simulink library "ConverterLibrary"  (R2026a)
settings: Solver=VariableStepAuto
undefined symbols (not defined in the file or in its folder): DiscIntNeverNeededParam, dspblkCoreblockFVToolHelper, gcbh, gridInverter
libraries: fl_lib x240, nesl_utility x221, ee_lib x208, slpidlib x28, eeGeneralControl x12, simulink x9, eeTransforms x4, simulink_extras x1, eePowerMeasurement x1
(part 15 of 30)

== system ConverterLibrary/Controller/Inverter-Based Resources/Grid-Forming Converter Controller/Grid Voltage Reactive Power Support/Modifying Reactive Power Reference/Changing the Power Reference/ActivePowerReference ==
  note: Ensure Pref sign is maintained
  Id : Inport
  Vd : Inport  Port=2
  Pref : Inport  Port=3
  Abs1 : Abs  SaturateOnIntegerOverflow=off
  Abs2 : Abs  SaturateOnIntegerOverflow=off
  Min : MinMax  Inputs=2
  Product : Product
  Product2 : Product
  Saturation : Saturate  UpperLimit=1  LowerLimit=-1
  Sign : Signum
  PrefNew : Outport
  wires:
  Saturation/1 -> PrefNew/1
  Vd/1 -> Product/2
  Abs2/1 -> Min/1
  Product2/1 -> Saturation/1
  Min/1 -> Product2/1
  Product/1 -> Abs2/1
  Abs1/1 -> Min/2
  Sign/1 -> Product2/2
  Id/1 -> Product/1
  Pref/1 -> Sign/1, Abs1/1

== system ConverterLibrary/Controller/Inverter-Based Resources/Grid-Forming Converter Controller/Grid Voltage Reactive Power Support/Modifying Reactive Power Reference/Changing the Power Reference/Estimate Id for Given Iq ==
  Iq : Inport
  Add Constant1 : Bias  Bias=1  SaturateOnIntegerOverflow=off
  Gain : Gain  Gain=-1
  Gain3 : Gain  Gain=0.9
  Sqrt : Sqrt
  Square : Math  Operator=square
  Id : Outport
  wires:
  Iq/1 -> Square/1
  Add Constant1/1 -> Sqrt/1
  Sqrt/1 -> Gain3/1
  Gain/1 -> Add Constant1/1
  Gain3/1 -> Id/1
  Square/1 -> Gain/1

== system ConverterLibrary/Controller/Inverter-Based Resources/Grid-Forming Converter Controller/Grid Voltage Reactive Power Support/Modifying Reactive Power Reference/Changing the Power Reference/EstimateIqForReactivePower ==
  note: Computing minimum reactive current as per GC0137
  Vmin : Inport
  Vd : Inport  Port=2
  Vs : Inport  Port=3
  Abs : Abs  SaturateOnIntegerOverflow=off
  Add : Sum
  Add Constant : Bias  Bias=1  SaturateOnIntegerOverflow=off
  GC0137 line slope : Gain  Gain=-1.4578
  Low Voltage Support : Subsystem
  Saturation : Saturate  UpperLimit=1  LowerLimit=0
  Iq : Outport
  wires:
  Low Voltage Support/1(Iqsupport) -> Add/1
  Vd/1 -> Low Voltage Support/2(Vd)
  Vmin/1 -> Low Voltage Support/1(Vin)
  Add Constant/1 -> Add/2
  Saturation/1 -> Iq/1
  Add/1 -> Saturation/1
  Vs/1 -> Abs/1
  GC0137 line slope/1 -> Add Constant/1
  Abs/1 -> GC0137 line slope/1

== system ConverterLibrary/Controller/Inverter-Based Resources/Grid-Forming Converter Controller/Grid Voltage Reactive Power Support/Modifying Reactive Power Reference/Changing the Power Reference/ReactivePowerReference ==
  Vd : Inport
  Iq : Inport  Port=2
  Compute Power : Product
  Constant : Constant  Value=0.3
  Gain2 : Gain  Gain=1.05
  Switch : Switch  Criteria=u2 > Threshold  Threshold=0.3  SaturateOnIntegerOverflow=off  InputSameDT=off
  QrefNew : Outport
  wires:
  Switch/1 -> Compute Power/1
  Vd/1 -> Switch/1, Switch/2
  Iq/1 -> Gain2/1
  Constant/1 -> Switch/3
  Gain2/1 -> Compute Power/2
  Compute Power/1 -> QrefNew/1

== system ConverterLibrary/Controller/Inverter-Based Resources/Grid-Forming Converter Controller/Measurement/Frequency Measurement/Frequency Measurement/If Action Subsystem ==
  V : Inport
  Time : Inport  Port=2
  Action Port : ActionPort
  Constant1 : Constant  Value=initialFrequency
  Delay : Delay  DelayLength=1
  Delay1 : Delay  DelayLength=1
  Frequency estimation : Subsystem  TreatAsAtomicUnit=on
  Hit Crossing : HitCross
  Switch : Switch  Criteria=u2 > Threshold  Threshold=1  SaturateOnIntegerOverflow=off  InputSameDT=off
  Freq : Outport
  wires:
  Switch/1 -> Freq/1
  Constant1/1 -> Switch/3
  Frequency estimation/1(f) -> Switch/1
  Time/1 -> Frequency estimation/3(k), Delay1/1, Switch/2
  Delay/1 -> Frequency estimation/2(sk-1)
  Hit Crossing/1 -> Frequency estimation/Trigger
  Delay1/1 -> Frequency estimation/4(k-1)
  V/1 -> Hit Crossing/1, Frequency estimation/1(sk), Delay/1

== system ConverterLibrary/Controller/Inverter-Based Resources/Grid-Forming Converter Controller/Measurement/Frequency Measurement/Frequency Measurement/If Action Subsystem1 ==
  Action Port : ActionPort
  Constant1 : Constant  Value=initialFrequency
  Out1 : Outport
  wires:
  Constant1/1 -> Out1/1

== system ConverterLibrary/Controller/Inverter-Based Resources/Grid-Forming Converter Controller/Measurement/Frequency Measurement/Frequency Measurement/Postive Sequence ==
  abc : Inport
  Complex to Real-Imag : ComplexToRealImag
  Demux : Demux  Outputs=3
  Symmetrical-Components Transform : eeTransforms/Symmetrical-Components Transform  PowerInvariant=off
      settings: LibrarySourceBlock=|
      | ee_sl_lib/Mathematical
      | Transforms/Symmetrical-Components
      | Transform
  Terminator : Terminator
  Terminator1 : Terminator
  Terminator2 : Terminator
  Transpose : Math  Operator=transpose
  posSeq : Outport
  wires:
  Demux/3 -> Terminator2/1
  Demux/2 -> Terminator1/1
  Complex to Real-Imag/2 -> Terminator/1
  abc/1 -> Transpose/1
  Demux/1 -> Complex to Real-Imag/1
  Complex to Real-Imag/1 -> posSeq/1
  Symmetrical-Components Transform/1 -> Demux/1
  Transpose/1 -> Symmetrical-Components Transform/1

== system ConverterLibrary/Controller/Inverter-Based Resources/Grid-Forming Converter Controller/Power Control/ActivePowerControl/vsmControl/Damping Frequency ==
  fref : Inport
  ConstantFreqReference : Subsystem  VariantControl=constFreq
  WithFrequencyMeasurement : Subsystem  VariantControl=freqMeas
  fmeas : Outport

== system ConverterLibrary/Controller/Non-Isolated DC-DC Converters/Non-Isolated DC-DC Controller/Loop Structure/DoubleLoop/Current Controller/PIContinuous ==
  error : Inport
  up : Inport  Port=2
  lo : Inport  Port=3
  PI Controller : slpidlib/PID Controller  Controller=PI  Form=Parallel  TimeDomain=Continuous-time  UseExternalTs=off  SampleTime=-1  IntegratorMethod=Forward Euler  FilterMethod=Forward Euler  ControllerParametersSource=internal  P=KpCurrent  I=KiCurrent  UseKiTs=off  D=0  UseExternalDerivativeSource=off  N=100  UseFilter=on  TunerSelectOption=Transfer Function Based (PID Tuner App)  InitialConditionSource=internal  InitialConditionForIntegrator=0  InitialConditionForFilter=0  DifferentiatorICPrevScaledInput=0  ExternalReset=none  TrackingMode=off  Kt=1  LimitOutput=on  SatLimitsSource=external  UpperSaturationLimit=1  LowerSaturationLimit=-1  LinearizeAsGain=on  AntiWindupMode=clamping  Kb=1  LimitIntegrator=on  UpperIntegratorSaturationLimit=dutyTrimSpan  LowerIntegratorSaturationLimit=-dutyTrimSpan  POutMin=[]  POutMax=[]  IOutMin=[]  IOutMax=[]  DOutMin=[]  DOutMax=[]  NOutMin=[]  NOutMax=[]  SumOutMin=[]  SumOutMax=[]  SaturationOutMin=[]  SaturationOutMax=[]  PParamMin=[]  PParamMax=[]  IParamMin=[]  IParamMax=[]  DParamMin=[]  DParamMax=[]  NParamMin=[]  NParamMax=[]  KbParamMin=[]  KbParamMax=[]  KtParamMin=[]  KtParamMax=[]  KbOutMin=[]  KbOutMax=[]  KtOutMin=[]  KtOutMax=[]  IntegratorOutMin=[]  IntegratorOutMax=[]  FilterOutMin=[]  FilterOutMax=[]  SumI1OutMin=[]  SumI1OutMax=[]  SumI2OutMin=[]  SumI2OutMax=[]  SumI3OutMin=[]  SumI3OutMax=[]  SumI4OutMin=[]  SumI4OutMax=[]  SumDOutMin=[]  SumDOutMax=[]  DifferentiatorOutMin=[]  DifferentiatorOutMax=[]  FilterDiffOutCoefMin=[]  FilterDiffOutCoefMax=[]  ReciprocalOutMin=[]  ReciprocalOutMax=[]  SumDenOutMin=[]  SumDenOutMax=[]  SumNumOutMin=[]  SumNumOutMax=[]  DivideOutMin=[]  DivideOutMax=[]  UdiffTsProdOutMin=[]  UdiffTsProdOutMax=[]  NTsProdOutMin=[]  NTsProdOutMax=[]  UintegralTsProdOutMin=[]  UintegralTsProdOutMax=[]  UngainTsProdOutMin=[]  UngainTsProdOutMax=[]  ClampingZeroOutDataTypeStr=Inherit: Inherit via back propagation  ClampingZeroOutMin=[]  ClampingZeroOutMax=[]  FilterDenConstantOutDataTypeStr=Inherit: Inherit via back propagation  FilterDenConstantOutMin=[]  FilterDenConstantOutMax=[]  PCopyOutDataTypeStr=Inherit: Inherit via back propagation  PCopyOutMin=[]  PCopyOutMax=[]  NCopyOutDataTypeStr=Inherit: Inherit via back propagation  NCopyOutMin=[]  NCopyOutMax=[]  IntegratorContinuousStateAttributes=''  IntegratorStateMustResolveToSignalObject=off  IntegratorRTWStateStorageClass=Auto  FilterContinuousStateAttributes=''  FilterStateMustResolveToSignalObject=off  FilterRTWStateStorageClass=Auto  ParallelPVariant=InternalParameters  IdealPVariant=Disabled  IVariant=InternalParameters  DVariant=Disabled  IntegratorVariant=Continuous  SatVariant=External  AWVariant=ContClampingParallel  PCopyVariant=Disabled  TRVariant=Disabled  FdbkBlocksVariant=Forward  IdealPFdbkVariant=Disabled  SatFdbkVariant=Disabled  DerivativeFilterVariant=Disabled  NVariant=Disabled  NCopyVariant=Disabled_SignalSpec  FilterICVariant=Disabled  IntegratorICVariant=InternalICs  ExternalResetVariant=Disabled  TRSumVariant=Passthrough  SumFdbkVariant=Disabled  SumVariant=Sum_PI  TsampFilterVariant=InternalTs  TsampNgainVariant=Passthrough  TsampIntegralVariant=Disabled_SignalSpec  ExternalSaturationOutDataTypeStr=Inherit: Same as second input  DerivativeSourceVariant=Disabled  PreIntVariant=InternalPreInt
  vc : Outport
  wires:
  error/1 -> PI Controller/1
  up/1 -> PI Controller/2
  lo/1 -> PI Controller/3
  PI Controller/1 -> vc/1

== system ConverterLibrary/Controller/Non-Isolated DC-DC Converters/Non-Isolated DC-DC Controller/Loop Structure/DoubleLoop/Current Controller/PIDiscrete ==
  error : Inport
  up : Inport  Port=2
  lo : Inport  Port=3
  PI Controller : slpidlib/PID Controller  Controller=PI  Form=Parallel  TimeDomain=Discrete-time  UseExternalTs=off  SampleTime=TsCurrent  IntegratorMethod=Backward Euler  FilterMethod=Forward Euler  ControllerParametersSource=internal  P=KpCurrent  I=KiCurrent  UseKiTs=off  D=0  UseExternalDerivativeSource=off  N=100  UseFilter=on  TunerSelectOption=Transfer Function Based (PID Tuner App)  InitialConditionSource=internal  InitialConditionForIntegrator=0  InitialConditionForFilter=0  DifferentiatorICPrevScaledInput=0  ExternalReset=none  TrackingMode=off  Kt=1  LimitOutput=on  SatLimitsSource=external  UpperSaturationLimit=1  LowerSaturationLimit=-1  LinearizeAsGain=on  AntiWindupMode=clamping  Kb=1  LimitIntegrator=on  UpperIntegratorSaturationLimit=dutyTrimSpan  LowerIntegratorSaturationLimit=-dutyTrimSpan  POutMin=[]  POutMax=[]  IOutMin=[]  IOutMax=[]  DOutMin=[]  DOutMax=[]  NOutMin=[]  NOutMax=[]  SumOutMin=[]  SumOutMax=[]  SaturationOutMin=[]  SaturationOutMax=[]  PParamMin=[]  PParamMax=[]  IParamMin=[]  IParamMax=[]  DParamMin=[]  DParamMax=[]  NParamMin=[]  NParamMax=[]  KbParamMin=[]  KbParamMax=[]  KtParamMin=[]  KtParamMax=[]  KbOutMin=[]  KbOutMax=[]  KtOutMin=[]  KtOutMax=[]  IntegratorOutMin=[]  IntegratorOutMax=[]  FilterOutMin=[]  FilterOutMax=[]  SumI1OutMin=[]  SumI1OutMax=[]  SumI2OutMin=[]  SumI2OutMax=[]  SumI3OutMin=[]  SumI3OutMax=[]  SumI4OutMin=[]  SumI4OutMax=[]  SumDOutMin=[]  SumDOutMax=[]  DifferentiatorOutMin=[]  DifferentiatorOutMax=[]  FilterDiffOutCoefMin=[]  FilterDiffOutCoefMax=[]  ReciprocalOutMin=[]  ReciprocalOutMax=[]  SumDenOutMin=[]  SumDenOutMax=[]  SumNumOutMin=[]  SumNumOutMax=[]  DivideOutMin=[]  DivideOutMax=[]  UdiffTsProdOutMin=[]  UdiffTsProdOutMax=[]  NTsProdOutMin=[]  NTsProdOutMax=[]  UintegralTsProdOutMin=[]  UintegralTsProdOutMax=[]  UngainTsProdOutMin=[]  UngainTsProdOutMax=[]  ClampingZeroOutDataTypeStr=Inherit: Inherit via back propagation  ClampingZeroOutMin=[]  ClampingZeroOutMax=[]  FilterDenConstantOutDataTypeStr=Inherit: Inherit via back propagation  FilterDenConstantOutMin=[]  FilterDenConstantOutMax=[]  PCopyOutDataTypeStr=Inherit: Inherit via back propagation  PCopyOutMin=[]  PCopyOutMax=[]  NCopyOutDataTypeStr=Inherit: Inherit via back propagation  NCopyOutMin=[]  NCopyOutMax=[]  IntegratorContinuousStateAttributes=''  IntegratorStateMustResolveToSignalObject=off  IntegratorRTWStateStorageClass=Auto  FilterContinuousStateAttributes=''  FilterStateMustResolveToSignalObject=off  FilterRTWStateStorageClass=Auto  ParallelPVariant=InternalParameters  IdealPVariant=Disabled  IVariant=InternalParameters  DVariant=Disabled  IntegratorVariant=Discrete  SatVariant=External  AWVariant=DiscClampingParallel  PCopyVariant=Disabled  TRVariant=Disabled  FdbkBlocksVariant=Feedback  IdealPFdbkVariant=Passthrough  SatFdbkVariant=Passthrough  DerivativeFilterVariant=Disabled  NVariant=Disabled  NCopyVariant=Disabled_SignalSpec  FilterICVariant=Disabled  IntegratorICVariant=InternalICs  ExternalResetVariant=Disabled  TRSumVariant=Passthrough  SumFdbkVariant=Enabled  SumVariant=Sum_PI  TsampFilterVariant=InternalTs  TsampNgainVariant=Passthrough  TsampIntegralVariant=Disabled_SignalSpec  ExternalSaturationOutDataTypeStr=Inherit: Same as second input  DerivativeSourceVariant=Disabled  PreIntVariant=InternalPreInt
  vc : Outport
  wires:
  error/1 -> PI Controller/1
  up/1 -> PI Controller/2
  PI Controller/1 -> vc/1
  lo/1 -> PI Controller/3

== system ConverterLibrary/Controller/Non-Isolated DC-DC Converters/Non-Isolated DC-DC Controller/Output Mode/PWMSignal/Half Bridge PWM Generator/Leg Gate Logic ==
  Ton : Inport
  Toff : Inport  Port=2
  S : Inport  Port=3
  After Turn Off : RelationalOperator
  After Turn On : RelationalOperator
  Pulse Window : Logic  Operator=XOR
  To Double : DataTypeConversion  OutDataTypeStr=double
  gates : Outport
  wires:
  Ton/1 -> After Turn On/2
  Toff/1 -> After Turn Off/2
  S/1 -> After Turn Off/1, After Turn On/1
  After Turn On/1 -> Pulse Window/1
  After Turn Off/1 -> Pulse Window/2
  Pulse Window/1 -> To Double/1
  To Double/1 -> gates/1

== system ConverterLibrary/Controller/Non-Isolated DC-DC Converters/Non-Isolated DC-DC Controller/Output Mode/PWMSignal/Half Bridge PWM Generator/Ramp Mode ==
  Tsw : Inport
  FixedStep : Subsystem  VariantControl=FixedStep
  VariableStep : Subsystem  VariantControl=VariableStep
  S : Outport

== system ConverterLibrary/Controller/PWM Generators/CLLC PWM Generator/Synchronous Rectifier/Turn On Delay/Rectifier Ramp Mode/FixedStep ==
  rate : Inport
  Rectifier Delay Timer : DiscreteIntegrator  SampleTime=Ts  LimitOutput=on  UpperSaturationLimit=Tsr  LowerSaturationLimit=0  ICPrevOutput=DiscIntNeverNeededParam  ICPrevScaledInput=DiscIntNeverNeededParam
  S : Outport
  wires:
  rate/1 -> Rectifier Delay Timer/1
  Rectifier Delay Timer/1 -> S/1

== system ConverterLibrary/Controller/PWM Generators/CLLC PWM Generator/Synchronous Rectifier/Turn On Delay/Rectifier Ramp Mode/VariableStep ==
  rate : Inport
  Rectifier Delay Timer : Integrator  LimitOutput=on  UpperSaturationLimit=Tsr  LowerSaturationLimit=0
  S : Outport
  wires:
  rate/1 -> Rectifier Delay Timer/1
  Rectifier Delay Timer/1 -> S/1

== system ConverterLibrary/Controller/Power Factor Correction Converters/Boost PFC Controller/Output Mode/PWMSignal/Ramp Mode/FixedStep ==
  Tsw : Inport
  Initial Ramp Value : InitialCondition  Value=0
  Overshoot Residual : Sum  Inputs=-+
  Period Reached : RelationalOperator  Operator=>  ZeroCross=off
  Time Ramp : DiscreteIntegrator  ExternalReset=rising  InitialConditionSource=external  SampleTime=Ts  ShowStatePort=on  ICPrevOutput=DiscIntNeverNeededParam  ICPrevScaledInput=DiscIntNeverNeededParam
  Unit Rate : Constant
  S : Outport
  wires:
  Unit Rate/1 -> Time Ramp/1
  Period Reached/1 -> Time Ramp/2
  Time Ramp/1 -> S/1
  Tsw/1 -> Overshoot Residual/1, Period Reached/2
  Time Ramp/State -> Period Reached/1, Overshoot Residual/2
  Overshoot Residual/1 -> Initial Ramp Value/1
  Initial Ramp Value/1 -> Time Ramp/3

== system ConverterLibrary/Controller/Power Factor Correction Converters/Boost PFC Controller/Output Mode/PWMSignal/Ramp Mode/VariableStep ==
  Tsw : Inport
  Initial Ramp Value : InitialCondition  Value=0
  Overshoot Residual : Sum  Inputs=-+
  Period Reached : RelationalOperator  Operator=>
  Time Ramp : Integrator  ExternalReset=rising  InitialConditionSource=external  ShowStatePort=on
  Unit Rate : Constant
  S : Outport
  wires:
  Unit Rate/1 -> Time Ramp/1
  Period Reached/1 -> Time Ramp/2
  Time Ramp/1 -> S/1
  Tsw/1 -> Overshoot Residual/1, Period Reached/2
  Time Ramp/State -> Period Reached/1, Overshoot Residual/2
  Overshoot Residual/1 -> Initial Ramp Value/1
  Initial Ramp Value/1 -> Time Ramp/3

== system ConverterLibrary/Controller/Power Factor Correction Converters/Interleaved Boost PFC Controller/Output Mode/PWMSignal/Ramp Mode/FixedStep ==
  Tsw : Inport
  Initial Ramp Value : InitialCondition  Value=0
  Overshoot Residual : Sum  Inputs=-+
  Period Reached : RelationalOperator  Operator=>  ZeroCross=off
  Time Ramp : DiscreteIntegrator  ExternalReset=rising  InitialConditionSource=external  SampleTime=Ts  ShowStatePort=on  ICPrevOutput=DiscIntNeverNeededParam  ICPrevScaledInput=DiscIntNeverNeededParam
  Unit Rate : Constant
  S : Outport
  wires:
  Unit Rate/1 -> Time Ramp/1
  Period Reached/1 -> Time Ramp/2
  Time Ramp/1 -> S/1
  Tsw/1 -> Overshoot Residual/1, Period Reached/2
  Time Ramp/State -> Period Reached/1, Overshoot Residual/2
  Overshoot Residual/1 -> Initial Ramp Value/1
  Initial Ramp Value/1 -> Time Ramp/3

== system ConverterLibrary/Controller/Power Factor Correction Converters/Interleaved Boost PFC Controller/Output Mode/PWMSignal/Ramp Mode/VariableStep ==
  Tsw : Inport
  Initial Ramp Value : InitialCondition  Value=0
  Overshoot Residual : Sum  Inputs=-+
  Period Reached : RelationalOperator  Operator=>
  Time Ramp : Integrator  ExternalReset=rising  InitialConditionSource=external  ShowStatePort=on
  Unit Rate : Constant
  S : Outport
  wires:
  Unit Rate/1 -> Time Ramp/1
  Period Reached/1 -> Time Ramp/2
  Time Ramp/1 -> S/1
  Tsw/1 -> Overshoot Residual/1, Period Reached/2
  Time Ramp/State -> Period Reached/1, Overshoot Residual/2
  Overshoot Residual/1 -> Initial Ramp Value/1
  Initial Ramp Value/1 -> Time Ramp/3

== system ConverterLibrary/Controller/Power Factor Correction Converters/Totem-Pole Boost PFC Controller/Gate Logic/Slow Leg Complementary PWM/Ramp Mode/FixedStep ==
  rate : Inport
  Dead Time Timer : DiscreteIntegrator  SampleTime=(1e-8)  LimitOutput=on  UpperSaturationLimit=(slowLegTurnOnDelay)  LowerSaturationLimit=0  ICPrevOutput=DiscIntNeverNeededParam  ICPrevScaledInput=DiscIntNeverNeededParam
  S : Outport
  wires:
  rate/1 -> Dead Time Timer/1
  Dead Time Timer/1 -> S/1

== system ConverterLibrary/Controller/Power Factor Correction Converters/Totem-Pole Boost PFC Controller/Gate Logic/Slow Leg Complementary PWM/Ramp Mode/VariableStep ==
  rate : Inport
  Dead Time Timer : Integrator  LimitOutput=on  UpperSaturationLimit=(slowLegTurnOnDelay)  LowerSaturationLimit=0
  S : Outport
  wires:
  rate/1 -> Dead Time Timer/1
  Dead Time Timer/1 -> S/1

== system ConverterLibrary/Controller/Power Factor Correction Converters/Totem-Pole Boost PFC Controller/Output Mode/PWMSignal/Half Bridge PWM Generator/Leg Gate Logic ==
  Ton : Inport
  Toff : Inport  Port=2
  S : Inport  Port=3
  After Turn Off : RelationalOperator
  After Turn On : RelationalOperator
  Pulse Window : Logic  Operator=XOR
  To Double : DataTypeConversion  OutDataTypeStr=double
  gates : Outport
  wires:
  To Double/1 -> gates/1
  Pulse Window/1 -> To Double/1
  After Turn Off/1 -> Pulse Window/2
  After Turn On/1 -> Pulse Window/1
  S/1 -> After Turn On/1, After Turn Off/1
  Toff/1 -> After Turn Off/2
  Ton/1 -> After Turn On/2

== system ConverterLibrary/Controller/Power Factor Correction Converters/Totem-Pole Boost PFC Controller/Output Mode/PWMSignal/Half Bridge PWM Generator/Ramp Mode ==
  Tsw : Inport
  FixedStep : Subsystem  VariantControl=FixedStep
  VariableStep : Subsystem  VariantControl=VariableStep
  S : Outport

== system ConverterLibrary/Controller/Soft-Switching Converters/CLLC Controller/Gate Signal/CLLC PWM Generator/Primary Gate Signal/Leg Gate Logic ==
  Ton : Inport
  Toff : Inport  Port=2
  S : Inport  Port=3
  After Turn Off : RelationalOperator
  After Turn On : RelationalOperator
  Pulse Window : Logic  Operator=XOR
  To Double : DataTypeConversion  OutDataTypeStr=double
  gates : Outport
  wires:
  Ton/1 -> After Turn On/2
  Toff/1 -> After Turn Off/2
  S/1 -> After Turn Off/1, After Turn On/1
  After Turn On/1 -> Pulse Window/1
  After Turn Off/1 -> Pulse Window/2
  Pulse Window/1 -> To Double/1
  To Double/1 -> gates/1

== system ConverterLibrary/Controller/Soft-Switching Converters/CLLC Controller/Gate Signal/CLLC PWM Generator/Primary Gate Signal/Ramp Mode ==
  Tsw : Inport
  FixedStep : Subsystem  VariantControl=FixedStep
  VariableStep : Subsystem  VariantControl=VariableStep
  S : Outport

== system ConverterLibrary/Controller/Soft-Switching Converters/CLLC Controller/Gate Signal/CLLC PWM Generator/Synchronous Rectifier/Conduction Detect ==
  Isec : Inport
  Conduction Pair : Mux  Inputs=2
  Forward Conduction : RelationalOperator
  Forward Threshold : Constant  Value=Ith
  Rectifier Gate Map : Selector  InputPortWidth=2  IndexOptions=Index vector (dialog)  Indices=[1 2 2 1]  OutputSizes=1
  Reverse Conduction : RelationalOperator  Operator=<=
  Reverse Threshold : Constant  Value=-Ith
  permit : Outport
  wires:
  Isec/1 -> Forward Conduction/1, Reverse Conduction/1
  Forward Threshold/1 -> Forward Conduction/2
  Reverse Threshold/1 -> Reverse Conduction/2
  Forward Conduction/1 -> Conduction Pair/1
  Reverse Conduction/1 -> Conduction Pair/2
  Conduction Pair/1 -> Rectifier Gate Map/1
  Rectifier Gate Map/1 -> permit/1

== system ConverterLibrary/Controller/Soft-Switching Converters/CLLC Controller/Gate Signal/CLLC PWM Generator/Synchronous Rectifier/Region Select ==
  primaryGates : Inport
  fpu : Inport  Port=2
  permit : Inport  Port=3
  Above Resonance : Subsystem
  Below Resonance : Subsystem
  If : If  IfExpression=u1 <= (0.97)  ElseIfExpressions=u1 >= (1.03)  SampleTime=0
  Rectifier Gates : Merge  Inputs=3
  Within Band : Subsystem
  Gs : Outport
  wires:
  fpu/1 -> If/1
  If/1 -> Below Resonance/Action
  primaryGates/1 -> Below Resonance/1(primaryGates), Above Resonance/1(primaryGates), Within Band/1(primaryGates)
  permit/1 -> Below Resonance/2(permit), Above Resonance/2(permit), Within Band/2(permit)
  Below Resonance/1(Gs) -> Rectifier Gates/1
  If/2 -> Above Resonance/Action
  Above Resonance/1(Gs) -> Rectifier Gates/2
  If/3 -> Within Band/Action
  Within Band/1(Gs) -> Rectifier Gates/3
  Rectifier Gates/1 -> Gs/1

== system ConverterLibrary/Controller/Soft-Switching Converters/CLLC Controller/Gate Signal/CLLC PWM Generator/Synchronous Rectifier/Turn On Delay ==
  condition : Inport
  Delay Elapsed : RelationalOperator
  Delay Time : Constant  Value=(Tdead)
  Logic To Double : DataTypeConversion  OutDataTypeStr=double
  Rate Offset : Bias  Bias=-1
  Rate Swing : Gain  Gain=2
  Rectifier Gate Window : Logic
  Rectifier Ramp Mode : Subsystem  Variant=on  VariantControlMode=label  LabelModeActiveChoice=VariableStep
  Gs : Outport
  wires:
  condition/1 -> Logic To Double/1, Rectifier Gate Window/1
  Logic To Double/1 -> Rate Swing/1
  Rate Swing/1 -> Rate Offset/1
  Rate Offset/1 -> Rectifier Ramp Mode/1(rate)
  Rectifier Ramp Mode/1(S) -> Delay Elapsed/1
  Delay Time/1 -> Delay Elapsed/2
  Delay Elapsed/1 -> Rectifier Gate Window/2
  Rectifier Gate Window/1 -> Gs/1

== system ConverterLibrary/Controller/Soft-Switching Converters/CLLC Controller/Voltage Controller/If Action Subsystem1/Voltage PI/PIContinuous ==
  error : Inport
  PID Controller : slpidlib/PID Controller  Controller=PID  Form=Parallel  TimeDomain=Continuous-time  UseExternalTs=off  SampleTime=-1  IntegratorMethod=Forward Euler  FilterMethod=Forward Euler  ControllerParametersSource=internal  P=Kpv  I=Kiv  UseKiTs=off  D=Kid  UseExternalDerivativeSource=off  N=100  UseFilter=on  TunerSelectOption=Transfer Function Based (PID Tuner App)  InitialConditionSource=internal  InitialConditionForIntegrator=0  InitialConditionForFilter=0  DifferentiatorICPrevScaledInput=0  ExternalReset=none  TrackingMode=off  Kt=1  LimitOutput=on  SatLimitsSource=internal  UpperSaturationLimit=IdcMax  LowerSaturationLimit=IdcMin  LinearizeAsGain=on  AntiWindupMode=clamping  Kb=1  LimitIntegrator=on  UpperIntegratorSaturationLimit=IdcMax  LowerIntegratorSaturationLimit=IdcMin  POutMin=[]  POutMax=[]  IOutMin=[]  IOutMax=[]  DOutMin=[]  DOutMax=[]  NOutMin=[]  NOutMax=[]  SumOutMin=[]  SumOutMax=[]  SaturationOutMin=[]  SaturationOutMax=[]  PParamMin=[]  PParamMax=[]  IParamMin=[]  IParamMax=[]  DParamMin=[]  DParamMax=[]  NParamMin=[]  NParamMax=[]  KbParamMin=[]  KbParamMax=[]  KtParamMin=[]  KtParamMax=[]  KbOutMin=[]  KbOutMax=[]  KtOutMin=[]  KtOutMax=[]  IntegratorOutMin=[]  IntegratorOutMax=[]  FilterOutMin=[]  FilterOutMax=[]  SumI1OutMin=[]  SumI1OutMax=[]  SumI2OutMin=[]  SumI2OutMax=[]  SumI3OutMin=[]  SumI3OutMax=[]  SumI4OutMin=[]  SumI4OutMax=[]  SumDOutMin=[]  SumDOutMax=[]  DifferentiatorOutMin=[]  DifferentiatorOutMax=[]  FilterDiffOutCoefMin=[]  FilterDiffOutCoefMax=[]  ReciprocalOutMin=[]  ReciprocalOutMax=[]  SumDenOutMin=[]  SumDenOutMax=[]  SumNumOutMin=[]  SumNumOutMax=[]  DivideOutMin=[]  DivideOutMax=[]  UdiffTsProdOutMin=[]  UdiffTsProdOutMax=[]  NTsProdOutMin=[]  NTsProdOutMax=[]  UintegralTsProdOutMin=[]  UintegralTsProdOutMax=[]  UngainTsProdOutMin=[]  UngainTsProdOutMax=[]  ClampingZeroOutDataTypeStr=Inherit: Inherit via back propagation  ClampingZeroOutMin=[]  ClampingZeroOutMax=[]  FilterDenConstantOutDataTypeStr=Inherit: Inherit via back propagation  FilterDenConstantOutMin=[]  FilterDenConstantOutMax=[]  PCopyOutDataTypeStr=Inherit: Inherit via back propagation  PCopyOutMin=[]  PCopyOutMax=[]  NCopyOutDataTypeStr=Inherit: Inherit via back propagation  NCopyOutMin=[]  NCopyOutMax=[]  IntegratorContinuousStateAttributes=''  IntegratorStateMustResolveToSignalObject=off  IntegratorRTWStateStorageClass=Auto  FilterContinuousStateAttributes=''  FilterStateMustResolveToSignalObject=off  FilterRTWStateStorageClass=Auto  ParallelPVariant=InternalParameters  IdealPVariant=Disabled  IVariant=InternalParameters  DVariant=InternalParameters  IntegratorVariant=Continuous  SatVariant=Enabled  AWVariant=ContClampingParallel  PCopyVariant=Disabled  TRVariant=Disabled  FdbkBlocksVariant=Forward  IdealPFdbkVariant=Disabled  SatFdbkVariant=Disabled  DerivativeFilterVariant=ContFilter  NVariant=InternalParameters  NCopyVariant=Disabled  FilterICVariant=InternalICsFilter  IntegratorICVariant=InternalICs  ExternalResetVariant=Disabled  TRSumVariant=Passthrough  SumFdbkVariant=Disabled  SumVariant=Sum_PID  TsampFilterVariant=InternalTs  TsampNgainVariant=Passthrough  TsampIntegralVariant=Disabled_SignalSpec  ExternalSaturationOutDataTypeStr=Inherit: Same as second input  DerivativeSourceVariant=ErrorSignal  PreIntVariant=InternalPreInt
  vc : Outport
  wires:
  PID Controller/1 -> vc/1
  error/1 -> PID Controller/1

== system ConverterLibrary/Controller/Soft-Switching Converters/CLLC Controller/Voltage Controller/If Action Subsystem1/Voltage PI/PIDiscrete ==
  error : Inport
  PID Controller : slpidlib/PID Controller  Controller=PID  Form=Parallel  TimeDomain=Discrete-time  UseExternalTs=off  SampleTime=TsVoltage  IntegratorMethod=Forward Euler  FilterMethod=Forward Euler  ControllerParametersSource=internal  P=Kpv  I=Kiv  UseKiTs=off  D=Kid  UseExternalDerivativeSource=off  N=100  UseFilter=on  TunerSelectOption=Transfer Function Based (PID Tuner App)  InitialConditionSource=internal  InitialConditionForIntegrator=0  InitialConditionForFilter=0  DifferentiatorICPrevScaledInput=0  ExternalReset=none  TrackingMode=off  Kt=1  LimitOutput=on  SatLimitsSource=internal  UpperSaturationLimit=IdcMax  LowerSaturationLimit=IdcMin  LinearizeAsGain=on  AntiWindupMode=clamping  Kb=1  LimitIntegrator=on  UpperIntegratorSaturationLimit=IdcMax  LowerIntegratorSaturationLimit=IdcMin  POutMin=[]  POutMax=[]  IOutMin=[]  IOutMax=[]  DOutMin=[]  DOutMax=[]  NOutMin=[]  NOutMax=[]  SumOutMin=[]  SumOutMax=[]  SaturationOutMin=[]  SaturationOutMax=[]  PParamMin=[]  PParamMax=[]  IParamMin=[]  IParamMax=[]  DParamMin=[]  DParamMax=[]  NParamMin=[]  NParamMax=[]  KbParamMin=[]  KbParamMax=[]  KtParamMin=[]  KtParamMax=[]  KbOutMin=[]  KbOutMax=[]  KtOutMin=[]  KtOutMax=[]  IntegratorOutMin=[]  IntegratorOutMax=[]  FilterOutMin=[]  FilterOutMax=[]  SumI1OutMin=[]  SumI1OutMax=[]  SumI2OutMin=[]  SumI2OutMax=[]  SumI3OutMin=[]  SumI3OutMax=[]  SumI4OutMin=[]  SumI4OutMax=[]  SumDOutMin=[]  SumDOutMax=[]  DifferentiatorOutMin=[]  DifferentiatorOutMax=[]  FilterDiffOutCoefMin=[]  FilterDiffOutCoefMax=[]  ReciprocalOutMin=[]  ReciprocalOutMax=[]  SumDenOutMin=[]  SumDenOutMax=[]  SumNumOutMin=[]  SumNumOutMax=[]  DivideOutMin=[]  DivideOutMax=[]  UdiffTsProdOutMin=[]  UdiffTsProdOutMax=[]  NTsProdOutMin=[]  NTsProdOutMax=[]  UintegralTsProdOutMin=[]  UintegralTsProdOutMax=[]  UngainTsProdOutMin=[]  UngainTsProdOutMax=[]  ClampingZeroOutDataTypeStr=Inherit: Inherit via back propagation  ClampingZeroOutMin=[]  ClampingZeroOutMax=[]  FilterDenConstantOutDataTypeStr=Inherit: Inherit via back propagation  FilterDenConstantOutMin=[]  FilterDenConstantOutMax=[]  PCopyOutDataTypeStr=Inherit: Inherit via back propagation  PCopyOutMin=[]  PCopyOutMax=[]  NCopyOutDataTypeStr=Inherit: Inherit via back propagation  NCopyOutMin=[]  NCopyOutMax=[]  IntegratorContinuousStateAttributes=''  IntegratorStateMustResolveToSignalObject=off  IntegratorRTWStateStorageClass=Auto  FilterContinuousStateAttributes=''  FilterStateMustResolveToSignalObject=off  FilterRTWStateStorageClass=Auto  ParallelPVariant=InternalParameters  IdealPVariant=Disabled  IVariant=InternalParameters  DVariant=InternalParameters  IntegratorVariant=Discrete  SatVariant=Enabled  AWVariant=DiscClampingParallel  PCopyVariant=Disabled  TRVariant=Disabled  FdbkBlocksVariant=Forward  IdealPFdbkVariant=Disabled  SatFdbkVariant=Disabled  DerivativeFilterVariant=ForwardEulerFilter  NVariant=InternalParameters  NCopyVariant=Disabled  FilterICVariant=InternalICsFilter  IntegratorICVariant=InternalICs  ExternalResetVariant=Disabled  TRSumVariant=Passthrough  SumFdbkVariant=Disabled  SumVariant=Sum_PID  TsampFilterVariant=InternalTs  TsampNgainVariant=Passthrough  TsampIntegralVariant=Disabled_SignalSpec  ExternalSaturationOutDataTypeStr=Inherit: Same as second input  DerivativeSourceVariant=ErrorSignal  PreIntVariant=InternalPreInt
  vc : Outport
  wires:
  PID Controller/1 -> vc/1
  error/1 -> PID Controller/1

== system ConverterLibrary/Controller/Soft-Switching Converters/DAB Controller (SPS)/CC-CV Control/CC Mode/Controller/PIContinuous ==
  error : Inport
  PI Controller : slpidlib/PID Controller  Controller=PI  Form=Parallel  TimeDomain=Continuous-time  UseExternalTs=off  SampleTime=-1  IntegratorMethod=Forward Euler  FilterMethod=Forward Euler  ControllerParametersSource=internal  P=Kp  I=Ki  UseKiTs=off  D=0.01  UseExternalDerivativeSource=off  N=100  UseFilter=on  TunerSelectOption=Transfer Function Based (PID Tuner App)  InitialConditionSource=internal  InitialConditionForIntegrator=0  InitialConditionForFilter=0  DifferentiatorICPrevScaledInput=0  ExternalReset=none  TrackingMode=off  Kt=1  LimitOutput=on  SatLimitsSource=internal  UpperSaturationLimit=phaseShiftMax*0.98  LowerSaturationLimit=phaseShiftMin*0.98  LinearizeAsGain=on  AntiWindupMode=clamping  Kb=1  LimitIntegrator=on  UpperIntegratorSaturationLimit=phaseShiftMax*0.98  LowerIntegratorSaturationLimit=phaseShiftMin*0.98  POutMin=[]  POutMax=[]  IOutMin=[]  IOutMax=[]  DOutMin=[]  DOutMax=[]  NOutMin=[]  NOutMax=[]  SumOutMin=[]  SumOutMax=[]  SaturationOutMin=[]  SaturationOutMax=[]  PParamMin=[]  PParamMax=[]  IParamMin=[]  IParamMax=[]  DParamMin=[]  DParamMax=[]  NParamMin=[]  NParamMax=[]  KbParamMin=[]  KbParamMax=[]  KtParamMin=[]  KtParamMax=[]  KbOutMin=[]  KbOutMax=[]  KtOutMin=[]  KtOutMax=[]  IntegratorOutMin=[]  IntegratorOutMax=[]  FilterOutMin=[]  FilterOutMax=[]  SumI1OutMin=[]  SumI1OutMax=[]  SumI2OutMin=[]  SumI2OutMax=[]  SumI3OutMin=[]  SumI3OutMax=[]  SumI4OutMin=[]  SumI4OutMax=[]  SumDOutMin=[]  SumDOutMax=[]  DifferentiatorOutMin=[]  DifferentiatorOutMax=[]  FilterDiffOutCoefMin=[]  FilterDiffOutCoefMax=[]  ReciprocalOutMin=[]  ReciprocalOutMax=[]  SumDenOutMin=[]  SumDenOutMax=[]  SumNumOutMin=[]  SumNumOutMax=[]  DivideOutMin=[]  DivideOutMax=[]  UdiffTsProdOutMin=[]  UdiffTsProdOutMax=[]  NTsProdOutMin=[]  NTsProdOutMax=[]  UintegralTsProdOutMin=[]  UintegralTsProdOutMax=[]  UngainTsProdOutMin=[]  UngainTsProdOutMax=[]  ClampingZeroOutDataTypeStr=Inherit: Inherit via back propagation  ClampingZeroOutMin=[]  ClampingZeroOutMax=[]  FilterDenConstantOutDataTypeStr=Inherit: Inherit via back propagation  FilterDenConstantOutMin=[]  FilterDenConstantOutMax=[]  PCopyOutDataTypeStr=Inherit: Inherit via back propagation  PCopyOutMin=[]  PCopyOutMax=[]  NCopyOutDataTypeStr=Inherit: Inherit via back propagation  NCopyOutMin=[]  NCopyOutMax=[]  IntegratorContinuousStateAttributes=''  IntegratorStateMustResolveToSignalObject=off  IntegratorRTWStateStorageClass=Auto  FilterContinuousStateAttributes=''  FilterStateMustResolveToSignalObject=off  FilterRTWStateStorageClass=Auto  ParallelPVariant=InternalParameters  IdealPVariant=Disabled  IVariant=InternalParameters  DVariant=Disabled  IntegratorVariant=Continuous  SatVariant=Enabled  AWVariant=ContClampingParallel  PCopyVariant=Disabled  TRVariant=Disabled  FdbkBlocksVariant=Forward  IdealPFdbkVariant=Disabled  SatFdbkVariant=Disabled  DerivativeFilterVariant=Disabled  NVariant=Disabled  NCopyVariant=Disabled_SignalSpec  FilterICVariant=Disabled  IntegratorICVariant=InternalICs  ExternalResetVariant=Disabled  TRSumVariant=Passthrough  SumFdbkVariant=Disabled  SumVariant=Sum_PI  TsampFilterVariant=InternalTs  TsampNgainVariant=Passthrough  TsampIntegralVariant=Disabled_SignalSpec  ExternalSaturationOutDataTypeStr=Inherit: Same as second input  DerivativeSourceVariant=Disabled  PreIntVariant=InternalPreInt
  vc : Outport
  wires:
  PI Controller/1 -> vc/1
  error/1 -> PI Controller/1

== system ConverterLibrary/Controller/Soft-Switching Converters/DAB Controller (SPS)/CC-CV Control/CC Mode/Controller/PIDiscrete ==
  error : Inport
  PI Controller : slpidlib/PID Controller  Controller=PI  Form=Parallel  TimeDomain=Discrete-time  UseExternalTs=off  SampleTime=Ts  IntegratorMethod=Forward Euler  FilterMethod=Forward Euler  ControllerParametersSource=internal  P=Kp  I=Ki  UseKiTs=off  D=0  UseExternalDerivativeSource=off  N=100  UseFilter=on  TunerSelectOption=Transfer Function Based (PID Tuner App)  InitialConditionSource=internal  InitialConditionForIntegrator=0  InitialConditionForFilter=0  DifferentiatorICPrevScaledInput=0  ExternalReset=none  TrackingMode=off  Kt=1  LimitOutput=on  SatLimitsSource=internal  UpperSaturationLimit=phaseShiftMax  LowerSaturationLimit=phaseShiftMin  LinearizeAsGain=on  AntiWindupMode=clamping  Kb=1  LimitIntegrator=on  UpperIntegratorSaturationLimit=phaseShiftMax  LowerIntegratorSaturationLimit=phaseShiftMin  POutMin=[]  POutMax=[]  IOutMin=[]  IOutMax=[]  DOutMin=[]  DOutMax=[]  NOutMin=[]  NOutMax=[]  SumOutMin=[]  SumOutMax=[]  SaturationOutMin=[]  SaturationOutMax=[]  PParamMin=[]  PParamMax=[]  IParamMin=[]  IParamMax=[]  DParamMin=[]  DParamMax=[]  NParamMin=[]  NParamMax=[]  KbParamMin=[]  KbParamMax=[]  KtParamMin=[]  KtParamMax=[]  KbOutMin=[]  KbOutMax=[]  KtOutMin=[]  KtOutMax=[]  IntegratorOutMin=[]  IntegratorOutMax=[]  FilterOutMin=[]  FilterOutMax=[]  SumI1OutMin=[]  SumI1OutMax=[]  SumI2OutMin=[]  SumI2OutMax=[]  SumI3OutMin=[]  SumI3OutMax=[]  SumI4OutMin=[]  SumI4OutMax=[]  SumDOutMin=[]  SumDOutMax=[]  DifferentiatorOutMin=[]  DifferentiatorOutMax=[]  FilterDiffOutCoefMin=[]  FilterDiffOutCoefMax=[]  ReciprocalOutMin=[]  ReciprocalOutMax=[]  SumDenOutMin=[]  SumDenOutMax=[]  SumNumOutMin=[]  SumNumOutMax=[]  DivideOutMin=[]  DivideOutMax=[]  UdiffTsProdOutMin=[]  UdiffTsProdOutMax=[]  NTsProdOutMin=[]  NTsProdOutMax=[]  UintegralTsProdOutMin=[]  UintegralTsProdOutMax=[]  UngainTsProdOutMin=[]  UngainTsProdOutMax=[]  ClampingZeroOutDataTypeStr=Inherit: Inherit via back propagation  ClampingZeroOutMin=[]  ClampingZeroOutMax=[]  FilterDenConstantOutDataTypeStr=Inherit: Inherit via back propagation  FilterDenConstantOutMin=[]  FilterDenConstantOutMax=[]  PCopyOutDataTypeStr=Inherit: Inherit via back propagation  PCopyOutMin=[]  PCopyOutMax=[]  NCopyOutDataTypeStr=Inherit: Inherit via back propagation  NCopyOutMin=[]  NCopyOutMax=[]  IntegratorContinuousStateAttributes=''  IntegratorStateMustResolveToSignalObject=off  IntegratorRTWStateStorageClass=Auto  FilterContinuousStateAttributes=''  FilterStateMustResolveToSignalObject=off  FilterRTWStateStorageClass=Auto  ParallelPVariant=InternalParameters  IdealPVariant=Disabled  IVariant=InternalParameters  DVariant=Disabled  IntegratorVariant=Discrete  SatVariant=Enabled  AWVariant=DiscClampingParallel  PCopyVariant=Disabled  TRVariant=Disabled  FdbkBlocksVariant=Forward  IdealPFdbkVariant=Disabled  SatFdbkVariant=Disabled  DerivativeFilterVariant=Disabled  NVariant=Disabled  NCopyVariant=Disabled_SignalSpec  FilterICVariant=Disabled  IntegratorICVariant=InternalICs  ExternalResetVariant=Disabled  TRSumVariant=Passthrough  SumFdbkVariant=Disabled  SumVariant=Sum_PI  TsampFilterVariant=InternalTs  TsampNgainVariant=Passthrough  TsampIntegralVariant=Disabled_SignalSpec  ExternalSaturationOutDataTypeStr=Inherit: Same as second input  DerivativeSourceVariant=Disabled  PreIntVariant=InternalPreInt
  vc : Outport
  wires:
  PI Controller/1 -> vc/1
  error/1 -> PI Controller/1

== system ConverterLibrary/Controller/Soft-Switching Converters/DAB Controller (SPS)/CC-CV Control/CV Mode/Voltage PI/PIContinuous ==
  error : Inport
  PI Controller : slpidlib/PID Controller  Controller=PI  Form=Parallel  TimeDomain=Continuous-time  UseExternalTs=off  SampleTime=-1  IntegratorMethod=Forward Euler  FilterMethod=Forward Euler  ControllerParametersSource=internal  P=Kpv  I=Kiv  UseKiTs=off  D=0.01  UseExternalDerivativeSource=off  N=100  UseFilter=on  TunerSelectOption=Transfer Function Based (PID Tuner App)  InitialConditionSource=internal  InitialConditionForIntegrator=0  InitialConditionForFilter=0  DifferentiatorICPrevScaledInput=0  ExternalReset=none  TrackingMode=off  Kt=1  LimitOutput=on  SatLimitsSource=internal  UpperSaturationLimit=phaseShiftMax*0.98  LowerSaturationLimit=phaseShiftMin*0.98  LinearizeAsGain=on  AntiWindupMode=clamping  Kb=1  LimitIntegrator=on  UpperIntegratorSaturationLimit=phaseShiftMax*0.98  LowerIntegratorSaturationLimit=phaseShiftMin*0.98  POutMin=[]  POutMax=[]  IOutMin=[]  IOutMax=[]  DOutMin=[]  DOutMax=[]  NOutMin=[]  NOutMax=[]  SumOutMin=[]  SumOutMax=[]  SaturationOutMin=[]  SaturationOutMax=[]  PParamMin=[]  PParamMax=[]  IParamMin=[]  IParamMax=[]  DParamMin=[]  DParamMax=[]  NParamMin=[]  NParamMax=[]  KbParamMin=[]  KbParamMax=[]  KtParamMin=[]  KtParamMax=[]  KbOutMin=[]  KbOutMax=[]  KtOutMin=[]  KtOutMax=[]  IntegratorOutMin=[]  IntegratorOutMax=[]  FilterOutMin=[]  FilterOutMax=[]  SumI1OutMin=[]  SumI1OutMax=[]  SumI2OutMin=[]  SumI2OutMax=[]  SumI3OutMin=[]  SumI3OutMax=[]  SumI4OutMin=[]  SumI4OutMax=[]  SumDOutMin=[]  SumDOutMax=[]  DifferentiatorOutMin=[]  DifferentiatorOutMax=[]  FilterDiffOutCoefMin=[]  FilterDiffOutCoefMax=[]  ReciprocalOutMin=[]  ReciprocalOutMax=[]  SumDenOutMin=[]  SumDenOutMax=[]  SumNumOutMin=[]  SumNumOutMax=[]  DivideOutMin=[]  DivideOutMax=[]  UdiffTsProdOutMin=[]  UdiffTsProdOutMax=[]  NTsProdOutMin=[]  NTsProdOutMax=[]  UintegralTsProdOutMin=[]  UintegralTsProdOutMax=[]  UngainTsProdOutMin=[]  UngainTsProdOutMax=[]  ClampingZeroOutDataTypeStr=Inherit: Inherit via back propagation  ClampingZeroOutMin=[]  ClampingZeroOutMax=[]  FilterDenConstantOutDataTypeStr=Inherit: Inherit via back propagation  FilterDenConstantOutMin=[]  FilterDenConstantOutMax=[]  PCopyOutDataTypeStr=Inherit: Inherit via back propagation  PCopyOutMin=[]  PCopyOutMax=[]  NCopyOutDataTypeStr=Inherit: Inherit via back propagation  NCopyOutMin=[]  NCopyOutMax=[]  IntegratorContinuousStateAttributes=''  IntegratorStateMustResolveToSignalObject=off  IntegratorRTWStateStorageClass=Auto  FilterContinuousStateAttributes=''  FilterStateMustResolveToSignalObject=off  FilterRTWStateStorageClass=Auto  ParallelPVariant=InternalParameters  IdealPVariant=Disabled  IVariant=InternalParameters  DVariant=Disabled  IntegratorVariant=Continuous  SatVariant=Enabled  AWVariant=ContClampingParallel  PCopyVariant=Disabled  TRVariant=Disabled  FdbkBlocksVariant=Forward  IdealPFdbkVariant=Disabled  SatFdbkVariant=Disabled  DerivativeFilterVariant=Disabled  NVariant=Disabled  NCopyVariant=Disabled_SignalSpec  FilterICVariant=Disabled  IntegratorICVariant=InternalICs  ExternalResetVariant=Disabled  TRSumVariant=Passthrough  SumFdbkVariant=Disabled  SumVariant=Sum_PI  TsampFilterVariant=InternalTs  TsampNgainVariant=Passthrough  TsampIntegralVariant=Disabled_SignalSpec  ExternalSaturationOutDataTypeStr=Inherit: Same as second input  DerivativeSourceVariant=Disabled  PreIntVariant=InternalPreInt
  vc : Outport
  wires:
  error/1 -> PI Controller/1
  PI Controller/1 -> vc/1

== system ConverterLibrary/Controller/Soft-Switching Converters/DAB Controller (SPS)/CC-CV Control/CV Mode/Voltage PI/PIDiscrete ==
  error : Inport
  PI Controller : slpidlib/PID Controller  Controller=PI  Form=Parallel  TimeDomain=Discrete-time  UseExternalTs=off  SampleTime=Ts  IntegratorMethod=Forward Euler  FilterMethod=Forward Euler  ControllerParametersSource=internal  P=Kpv  I=Kiv  UseKiTs=off  D=0  UseExternalDerivativeSource=off  N=100  UseFilter=on  TunerSelectOption=Transfer Function Based (PID Tuner App)  InitialConditionSource=internal  InitialConditionForIntegrator=0  InitialConditionForFilter=0  DifferentiatorICPrevScaledInput=0  ExternalReset=none  TrackingMode=off  Kt=1  LimitOutput=on  SatLimitsSource=internal  UpperSaturationLimit=phaseShiftMax  LowerSaturationLimit=phaseShiftMin  LinearizeAsGain=on  AntiWindupMode=clamping  Kb=1  LimitIntegrator=on  UpperIntegratorSaturationLimit=phaseShiftMax  LowerIntegratorSaturationLimit=phaseShiftMin  POutMin=[]  POutMax=[]  IOutMin=[]  IOutMax=[]  DOutMin=[]  DOutMax=[]  NOutMin=[]  NOutMax=[]  SumOutMin=[]  SumOutMax=[]  SaturationOutMin=[]  SaturationOutMax=[]  PParamMin=[]  PParamMax=[]  IParamMin=[]  IParamMax=[]  DParamMin=[]  DParamMax=[]  NParamMin=[]  NParamMax=[]  KbParamMin=[]  KbParamMax=[]  KtParamMin=[]  KtParamMax=[]  KbOutMin=[]  KbOutMax=[]  KtOutMin=[]  KtOutMax=[]  IntegratorOutMin=[]  IntegratorOutMax=[]  FilterOutMin=[]  FilterOutMax=[]  SumI1OutMin=[]  SumI1OutMax=[]  SumI2OutMin=[]  SumI2OutMax=[]  SumI3OutMin=[]  SumI3OutMax=[]  SumI4OutMin=[]  SumI4OutMax=[]  SumDOutMin=[]  SumDOutMax=[]  DifferentiatorOutMin=[]  DifferentiatorOutMax=[]  FilterDiffOutCoefMin=[]  FilterDiffOutCoefMax=[]  ReciprocalOutMin=[]  ReciprocalOutMax=[]  SumDenOutMin=[]  SumDenOutMax=[]  SumNumOutMin=[]  SumNumOutMax=[]  DivideOutMin=[]  DivideOutMax=[]  UdiffTsProdOutMin=[]  UdiffTsProdOutMax=[]  NTsProdOutMin=[]  NTsProdOutMax=[]  UintegralTsProdOutMin=[]  UintegralTsProdOutMax=[]  UngainTsProdOutMin=[]  UngainTsProdOutMax=[]  ClampingZeroOutDataTypeStr=Inherit: Inherit via back propagation  ClampingZeroOutMin=[]  ClampingZeroOutMax=[]  FilterDenConstantOutDataTypeStr=Inherit: Inherit via back propagation  FilterDenConstantOutMin=[]  FilterDenConstantOutMax=[]  PCopyOutDataTypeStr=Inherit: Inherit via back propagation  PCopyOutMin=[]  PCopyOutMax=[]  NCopyOutDataTypeStr=Inherit: Inherit via back propagation  NCopyOutMin=[]  NCopyOutMax=[]  IntegratorContinuousStateAttributes=''  IntegratorStateMustResolveToSignalObject=off  IntegratorRTWStateStorageClass=Auto  FilterContinuousStateAttributes=''  FilterStateMustResolveToSignalObject=off  FilterRTWStateStorageClass=Auto  ParallelPVariant=InternalParameters  IdealPVariant=Disabled  IVariant=InternalParameters  DVariant=Disabled  IntegratorVariant=Discrete  SatVariant=Enabled  AWVariant=DiscClampingParallel  PCopyVariant=Disabled  TRVariant=Disabled  FdbkBlocksVariant=Forward  IdealPFdbkVariant=Disabled  SatFdbkVariant=Disabled  DerivativeFilterVariant=Disabled  NVariant=Disabled  NCopyVariant=Disabled_SignalSpec  FilterICVariant=Disabled  IntegratorICVariant=InternalICs  ExternalResetVariant=Disabled  TRSumVariant=Passthrough  SumFdbkVariant=Disabled  SumVariant=Sum_PI  TsampFilterVariant=InternalTs  TsampNgainVariant=Passthrough  TsampIntegralVariant=Disabled_SignalSpec  ExternalSaturationOutDataTypeStr=Inherit: Same as second input  DerivativeSourceVariant=Disabled  PreIntVariant=InternalPreInt
  vc : Outport
  wires:
  error/1 -> PI Controller/1
  PI Controller/1 -> vc/1

== system ConverterLibrary/Controller/Soft-Switching Converters/DAB Controller (SPS)/Output Mode/PWMSignal/Gate Signal Generator/Phase-Shifted Sawtooth ==
  S : Inport
  tPhase : Inport  Port=2
  Ts : Inport  Port=3
  Add : Sum
  Mod : Math  Operator=mod
  PS : Outport
  wires:
  S/1 -> Add/1
  Add/1 -> Mod/1
  Ts/1 -> Mod/2
  Mod/1 -> PS/1
  tPhase/1 -> Add/2

== system ConverterLibrary/Controller/Soft-Switching Converters/DAB Controller (SPS)/Output Mode/PWMSignal/Gate Signal Generator/Primary Bridge Gate ==
  S : Inport
  Ton : Inport  Port=2
  Toff : Inport  Port=3
  Demux : Demux  Outputs=3
  Logical Operator : Logic  Operator=XOR  AllPortsSameDT=off  OutDataTypeStr=boolean
  Logical Operator1 : Logic  Operator=XOR  AllPortsSameDT=off  OutDataTypeStr=boolean
  Logical Operator2 : Logic  Operator=XOR  AllPortsSameDT=off  OutDataTypeStr=boolean
  Logical Operator3 : Logic  Operator=NOT  AllPortsSameDT=off  OutDataTypeStr=boolean
  Mux : Mux
  Rate Transition : RateTransition
  Rate Transition1 : RateTransition
  Relational Operator : RelationalOperator  OutDataTypeStr=boolean  InputSameDT=off
  Relational Operator3 : RelationalOperator  OutDataTypeStr=boolean  InputSameDT=off
  G : Outport
  wires:
  Logical Operator2/1 -> Mux/2, Mux/3
  Relational Operator/1 -> Logical Operator/1
  S/1 -> Relational Operator3/1, Relational Operator/1
  Rate Transition1/1 -> Relational Operator3/2
  Relational Operator3/1 -> Logical Operator/2
  Rate Transition/1 -> Relational Operator/2
  Toff/1 -> Rate Transition1/1
  Ton/1 -> Rate Transition/1
  Logical Operator/1 -> Demux/1
  Demux/1 -> Logical Operator1/1, Logical Operator3/1
  Demux/2 -> Logical Operator1/2
  Demux/3 -> Logical Operator2/2
  Logical Operator3/1 -> Logical Operator2/1
  Logical Operator1/1 -> Mux/4, Mux/1
  Mux/1 -> G/1

== system ConverterLibrary/Controller/Soft-Switching Converters/DAB Controller (SPS)/Output Mode/PWMSignal/Gate Signal Generator/Sawtooth Time Generator ==
  Ts : Inport
  Add3 : Sum  Inputs=-+
  Constant2 : Constant
  Discrete-Time Integrator1 : DiscreteIntegrator  ExternalReset=rising  InitialConditionSource=external  SampleTime=-1  ShowStatePort=on  ICPrevOutput=DiscIntNeverNeededParam  ICPrevScaledInput=DiscIntNeverNeededParam
  Initial : InitialCondition  Value=0
  Relational Operator1 : RelationalOperator  Operator=>  OutDataTypeStr=boolean  InputSameDT=off
  TimeRamp : Outport
  wires:
  Relational Operator1/1 -> Discrete-Time Integrator1/2
  Constant2/1 -> Discrete-Time Integrator1/1
  Discrete-Time Integrator1/1 -> TimeRamp/1
  Ts/1 -> Add3/1, Relational Operator1/2
  Discrete-Time Integrator1/State -> Add3/2, Relational Operator1/1
  Add3/1 -> Initial/1
  Initial/1 -> Discrete-Time Integrator1/3

== system ConverterLibrary/Controller/Soft-Switching Converters/DAB Controller (SPS)/Output Mode/PWMSignal/Gate Signal Generator/Secondary Bridge Gate ==
  Ton : Inport
  Toff : Inport  Port=2
  S : Inport  Port=3
  Demux : Demux  Outputs=3
  Logical Operator : Logic  Operator=XOR  AllPortsSameDT=off  OutDataTypeStr=boolean
  Logical Operator1 : Logic  Operator=XOR  AllPortsSameDT=off  OutDataTypeStr=boolean
  Logical Operator2 : Logic  Operator=XOR  AllPortsSameDT=off  OutDataTypeStr=boolean
  Logical Operator3 : Logic  Operator=NOT  AllPortsSameDT=off  OutDataTypeStr=boolean
  Mux : Mux
  Rate Transition : RateTransition
  Rate Transition1 : RateTransition
  Relational Operator : RelationalOperator  OutDataTypeStr=boolean  InputSameDT=off
  Relational Operator3 : RelationalOperator  OutDataTypeStr=boolean  InputSameDT=off
  G : Outport
  wires:
  Logical Operator2/1 -> Mux/3, Mux/2
  Relational Operator/1 -> Logical Operator/1
  S/1 -> Relational Operator3/1, Relational Operator/1
  Rate Transition1/1 -> Relational Operator3/2
  Relational Operator3/1 -> Logical Operator/2
  Rate Transition/1 -> Relational Operator/2
  Toff/1 -> Rate Transition1/1
  Ton/1 -> Rate Transition/1
  Logical Operator/1 -> Demux/1
  Demux/1 -> Logical Operator1/1, Logical Operator3/1
  Demux/2 -> Logical Operator1/2
  Demux/3 -> Logical Operator2/2
  Logical Operator3/1 -> Logical Operator2/1
  Logical Operator1/1 -> Mux/1, Mux/4
  Mux/1 -> G/1

== system ConverterLibrary/Power Converter Plant/Non-Isolated DC-DC Converters/Non-Isolated DC-DC Converter/NonIsolatedDCDCVariant/Boost/Diode/IdealDiode ==
  Diode : fl_lib/Electrical/Electrical Elements/Diode  Vf=Vf_SI V  Ron=Rd_SI Ohm  Goff=Gd_SI 1/Ohm  i_specify=off  i_priority=None  i=0 A  i_nominal_specify=off  i_nominal_value=1  i_nominal_unit=A  v_specify=off  v_priority=None  v=0 V  v_nominal_specify=off  v_nominal_value=1  v_nominal_unit=V
  D : PMIOPort  Side=Left
  S : PMIOPort  Port=2  Side=Right
  connections:
  Diode/RConn1 -- S/RConn1
  D/RConn1 -- Diode/LConn1
